simulink library "simpleFuselage_lib"  (R2018b)
settings: Solver=VariableStepAuto  StartTime=0.0  StopTime=10.0  RelTol=1e-3
values from neighbouring files (symbols this model uses):
  simple_fuselage = simpleFuselageCreate('simpleFuselage_params_default',V)    [simpleFuselage_lib_example_init.m]
libraries: axes_transformation_lib x1
settings Model: Creator=Ybeyer  LastModifiedBy=yannic
settings SFSimCC: SimUseLocalCustomCode=off
settings RTWCC: RTWUseLocalCustomCode=off
settings CodeAppCC: StateflowObjectComments=on

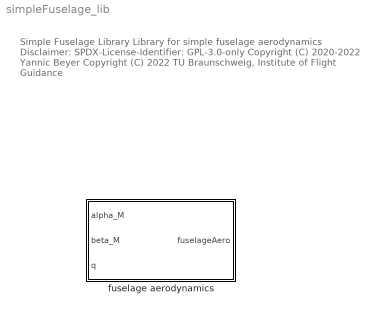
== system simpleFuselage_lib ==
  note: Simple Fuselage Library
      |
      | Library for simple fuselage aerodynamics
      |
      | Disclaimer:
      | SPDX-License-Identifier: GPL-3.0-only
      |
      | Copyright (C) 2020-2022 Yannic Beyer
      | Copyright (C) 2022 TU Braunschweig, Institute of Flight Guidance
  fuselage aerodynamics : Subsystem  mask{simple_fuselage=simple_fuselage}
      mask prompts: simple_fuselage "Simple fuselage struct"
      mask DialogControl DescGroupVar Prompt: Simple fuselage aerodynamics
      mask DialogControl DescTextVar Prompt: This block computes the aerodynamics of a fuselage at a reference point. It is a semi-empirical model based on basic literature.
      mask DialogControl Control2 Prompt: For more information take a look at the README:
      mask DialogControl Control3 Prompt: README
      mask DialogControl Control3 Callback: web('https://github.com/iff-gsc/ladac/-/blob/master/aerodynamics/simple_fuselage/README.md','-browser')
      mask DialogControl Control4 Prompt: To initialize a simple fuselage struct, please use the function simpleFuselageCreate.

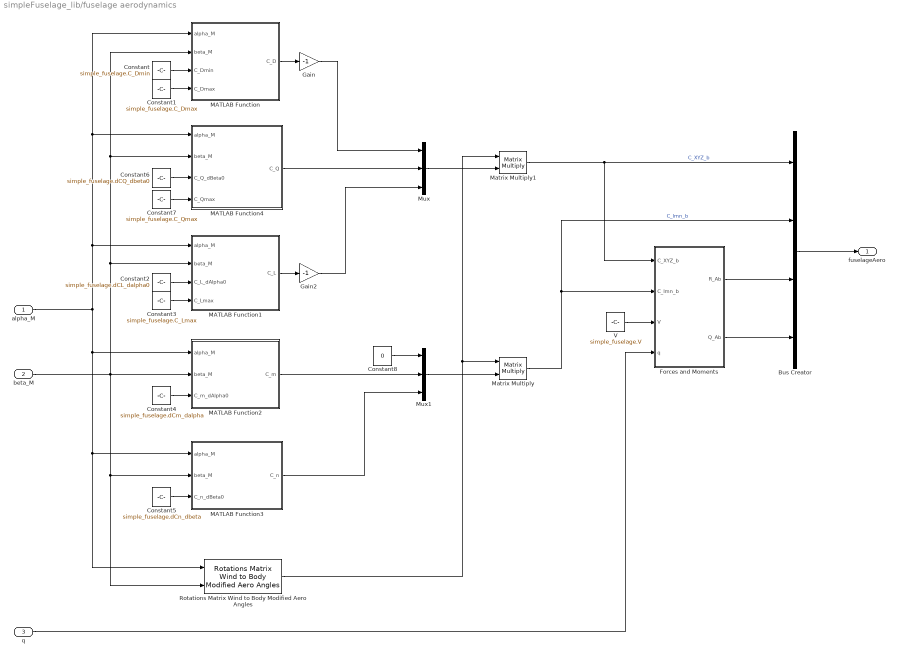
== system simpleFuselage_lib/fuselage aerodynamics ==
  alpha_M : Inport
  beta_M : Inport  Port=2
  q : Inport  Port=3
  Bus Creator : BusCreator  Inputs=4
  Constant : Constant  Value=simple_fuselage.C_Dmin
  Constant1 : Constant  Value=simple_fuselage.C_Dmax
  Constant2 : Constant  Value=simple_fuselage.dCL_dalpha0
  Constant3 : Constant  Value=simple_fuselage.C_Lmax
  Constant4 : Constant  Value=simple_fuselage.dCm_dalpha
  Constant5 : Constant  Value=simple_fuselage.dCn_dbeta
  Constant6 : Constant  Value=simple_fuselage.dCQ_dbeta0
  Constant7 : Constant  Value=simple_fuselage.C_Qmax
  Constant8 : Constant  Value=0
  Forces and Moments : MATLAB Function  TreatAsAtomicUnit=on
  Gain : Gain  Gain=-1
  Gain2 : Gain  Gain=-1
  MATLAB Function : MATLAB Function  TreatAsAtomicUnit=on
  MATLAB Function1 : MATLAB Function  TreatAsAtomicUnit=on
  MATLAB Function2 : MATLAB Function  TreatAsAtomicUnit=on
  MATLAB Function3 : MATLAB Function  TreatAsAtomicUnit=on
  MATLAB Function4 : MATLAB Function  TreatAsAtomicUnit=on
  Matrix Multiply : Product  Multiplication=Matrix(*)
  Matrix Multiply1 : Product  Multiplication=Matrix(*)
  Mux : Mux  Inputs=3
  Mux1 : Mux  Inputs=3
  Rotations Matrix Wind to Body Modified Aero Angles : axes_transformation_lib/Rotations Matrix Wind to Body Modified Aero Angles  SystemSampleTime=-1
      settings: SourceProductName=LADAC
  V : Constant  Value=simple_fuselage.V
  fuselageAero : Outport
  wires:
  q/1 -> Forces and Moments/4(q)
  Bus Creator/1 -> fuselageAero/1
  Forces and Moments/2(Q_Ab) -> Bus Creator/4
  Forces and Moments/1(R_Ab) -> Bus Creator/3
  V/1 -> Forces and Moments/3(V)
  Matrix Multiply1/1 -> Forces and Moments/1(C_XYZ_b), Bus Creator/1  "C_XYZ_b"
  Rotations Matrix Wind to Body Modified Aero Angles/1 -> Matrix Multiply/1, Matrix Multiply1/1
  Matrix Multiply/1 -> Forces and Moments/2(C_lmn_b), Bus Creator/2  "C_lmn_b"
  alpha_M/1 -> MATLAB Function2/1(alpha_M), MATLAB Function3/1(alpha_M), Rotations Matrix Wind to Body Modified Aero Angles/1, MATLAB Function1/1(alpha_M), MATLAB Function4/1(alpha_M), MATLAB Function/1(alpha_M)
  Gain2/1 -> Mux/3
  MATLAB Function4/1(C_Q) -> Mux/2
  Gain/1 -> Mux/1
  Mux1/1 -> Matrix Multiply/2
  Mux/1 -> Matrix Multiply1/2
  Constant8/1 -> Mux1/1
  MATLAB Function3/1(C_n) -> Mux1/3
  MATLAB Function2/1(C_m) -> Mux1/2
  MATLAB Function1/1(C_L) -> Gain2/1
  MATLAB Function/1(C_D) -> Gain/1
  Constant7/1 -> MATLAB Function4/4(C_Qmax)
  Constant6/1 -> MATLAB Function4/3(C_Q_dBeta0)
  Constant5/1 -> MATLAB Function3/3(C_n_dBeta0)
  Constant4/1 -> MATLAB Function2/3(C_m_dAlpha0)
  Constant3/1 -> MATLAB Function1/4(C_Lmax)
  Constant2/1 -> MATLAB Function1/3(C_L_dAlpha0)
  Constant1/1 -> MATLAB Function/4(C_Dmax)
  Constant/1 -> MATLAB Function/3(C_Dmin)
  beta_M/1 -> MATLAB Function2/2(beta_M), MATLAB Function3/2(beta_M), Rotations Matrix Wind to Body Modified Aero Angles/2, MATLAB Function1/2(beta_M), MATLAB Function4/2(beta_M), MATLAB Function/2(beta_M)

== matlab function simpleFuselage_lib/fuselage aerodynamics/MATLAB Function1 ==
  data: alpha_M input; C_L output; beta_M input; C_L_dAlpha0 input; C_Lmax input
function C_L = fcn( alpha_M, beta_M, C_L_dAlpha0, C_Lmax ) %#codegen

C_L = simpleFuselageCl( alpha_M, beta_M, C_L_dAlpha0, C_Lmax );

end

== matlab function simpleFuselage_lib/fuselage aerodynamics/MATLAB Function3 ==
  data: alpha_M input; C_n output; beta_M input; C_n_dBeta0 input
function C_n = fcn( alpha_M, beta_M, C_n_dBeta0 ) %#codegen

C_n = simpleFuselageCn( alpha_M, beta_M, C_n_dBeta0 );

end

== matlab function simpleFuselage_lib/fuselage aerodynamics/MATLAB Function ==
  data: alpha_M input; C_D output; beta_M input; C_Dmin input; C_Dmax input
function C_D = fcn( alpha_M, beta_M, C_Dmin, C_Dmax ) %#codegen

C_D = simpleFuselageCd( alpha_M, beta_M, C_Dmin, C_Dmax );

end

== matlab function simpleFuselage_lib/fuselage aerodynamics/MATLAB Function2 ==
  data: alpha_M input; C_m output; beta_M input; C_m_dAlpha0 input
function C_m = fcn( alpha_M, beta_M, C_m_dAlpha0 ) %#codegen

C_m = simpleFuselageCm( alpha_M, beta_M, C_m_dAlpha0 );

end

== matlab function simpleFuselage_lib/fuselage aerodynamics/MATLAB Function4 ==
  data: alpha_M input; C_Q output; beta_M input; C_Q_dBeta0 input; C_Qmax input
function C_Q = fcn( alpha_M, beta_M, C_Q_dBeta0, C_Qmax ) %#codegen

C_Q = simpleFuselageCq( alpha_M, beta_M, C_Q_dBeta0, C_Qmax );

end

== matlab function simpleFuselage_lib/fuselage aerodynamics/Forces and Moments ==
  data: C_XYZ_b input; R_Ab output; C_lmn_b input; V input; Q_Ab output; q input
function [ R_Ab, Q_Ab ] = fcn(C_XYZ_b, C_lmn_b, V, q) %#codegen

V = max(0,V);

R_Ab = C_XYZ_b * V^(2/3) * q;

Q_Ab = C_lmn_b * V * q;

end
